simulink model "sf_fixpt_conversion"  (R2025b)
settings: Solver=VariableStepAuto  StartTime=0.0  StopTime=10.0  RelTol=1e-3
settings Model: Creator=The MathWorks, Inc.  LastModifiedBy=The MathWorks, Inc.
settings SolverCC: AlgebraicLoopSolver=TrustRegion
settings DataIOCC: ReturnWorkspaceOutputs=off
settings OptimizationCC: ReuseModelBlockBuffer=off
settings DebuggingCC: UnconnectedInputMsg=warning  UnconnectedOutputMsg=warning  UnconnectedLineMsg=warning  ArithmeticOperatorsInVariantConditions=warning
settings ModelReferenceCC: EnableRefExpFcnMdlSchedulingChecks=on
settings RTWCC: GPUComputeCapability=3.5  DLArmComputeVersion=19.05

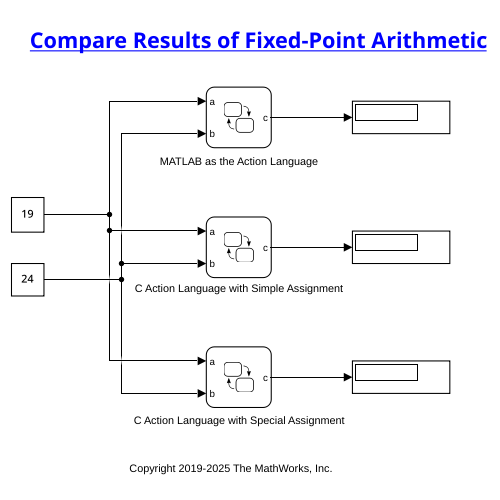
[thumbnail: Simulink's stored preview of the top-level diagram]
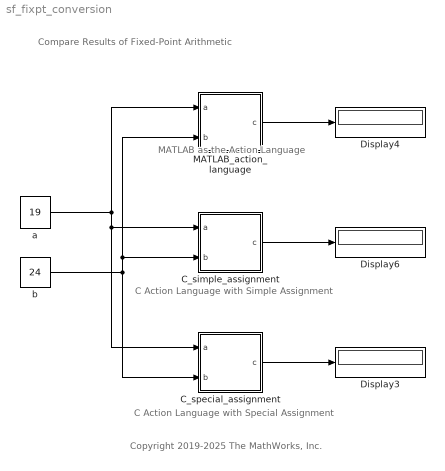
== system sf_fixpt_conversion ==
  note: Copyright 2019-2025 The MathWorks, Inc.
  note: C Action Language with Special Assignment
  note: C Action Language with Simple Assignment
  note: MATLAB as the Action Language
  note: Compare Results of Fixed-Point Arithmetic
  C_simple_assignment : Stateflow chart  TreatAsAtomicUnit=on
  C_special_assignment : Stateflow chart  TreatAsAtomicUnit=on
  Display3 : Display
  Display4 : Display
  Display6 : Display
  MATLAB_action_language : Stateflow chart  TreatAsAtomicUnit=on
  a : Constant  Value=19  OutDataTypeStr=fixdt(1,16,1)
  b : Constant  Value=24  OutDataTypeStr=fixdt(1,16,1)
  wires:
  a/1 -> C_special_assignment/1(a), C_simple_assignment/1(a), MATLAB_action_language/1(a)
  b/1 -> MATLAB_action_language/2(b), C_simple_assignment/2(b), C_special_assignment/2(b)
  MATLAB_action_language/1(c) -> Display4/1
  C_simple_assignment/1(c) -> Display6/1
  C_special_assignment/1(c) -> Display3/1

== stateflow chart sf_fixpt_conversion/C_special_assignment ==
  state A1
    % C as the action language
    % Special assignment operation (:=)
    c := a/b;
  (default) -> A1
  data: a input fixdt(1,16,1); b input fixdt(1,16,1); c output fixdt(1,16,1) size=1

== stateflow chart sf_fixpt_conversion/MATLAB_action_language ==
  state A
    % MATLAB as the action language
    c = cast(a/b,'like',c);
  (default) -> A
  data: a input fixdt(1,16,1); b input fixdt(1,16,1); c output fixdt(1,16,1) size=1

== stateflow chart sf_fixpt_conversion/C_simple_assignment ==
  state A1
    % C as the action language
    % Simple assignment operation (=)
    c = a/b;
  (default) -> A1
  data: a input fixdt(1,16,1); b input fixdt(1,16,1); c output fixdt(1,16,1) size=1
